simulink model "BMS_Controller"  (R2025b)
settings: Solver=FixedStepDiscrete  StartTime=0.0  StopTime=10.0  FixedStep=Ts  RelTol=1e-3
InitFcn:
  | init_BMS
undefined symbols (not defined in the file): I_charge_OC_release_A, I_charge_OC_trip_A, I_discharge_OC_release_A, I_discharge_OC_trip_A, Q_est_cell_Ah, SOC0_est_pack, T_charge_high_release_C, T_charge_high_trip_C, T_charge_low_release_C, T_charge_low_trip_C, T_discharge_high_release_C, T_discharge_high_trip_C, T_discharge_low_release_C, T_discharge_low_trip_C, Ts, V_cell_OV_release_V, V_cell_OV_trip_V, V_cell_UV_release_V, V_cell_UV_trip_V
libraries: simulink x7
settings Model: Creator=Khadija  LastModifiedBy=Khadija
settings OptimizationCC: DefaultParameterBehavior=Inlined  EnhancedBackFolding=on  PassReuseOutputArgsAs=Individual arguments  ZeroExternalMemoryAtStartup=off  ZeroInternalMemoryAtStartup=off  OptimizeBlockOrder=speed  DifferentSizesBufferReuse=on  OptimizationCustomize=off  EfficientTunableParamExpr=on
settings DebuggingCC: ParameterTunabilityLossMsg=error
settings SFSimCC: MATLABDynamicMemAlloc=off
settings RTWCC: SystemTargetFile=ert.tlc  TemplateMakefile=ert_default_tmf  Description=Embedded Coder
settings CodeAppCC: ForceParamTrailComments=on  IgnoreCustomStorageClasses=off  OperatorAnnotations=on  SimulinkDataObjDesc=on  SFDataObjDesc=on  InsertBlockDesc=on
settings ERTTargetCC: ERTCustomFileTemplate=example_file_process.tlc  TargetLangStandard=C99 (ISO)  GenerateSampleERTMain=on

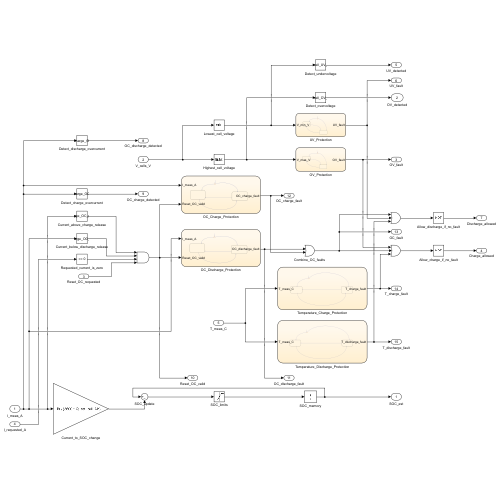
[thumbnail: Simulink's stored preview of the top-level diagram]
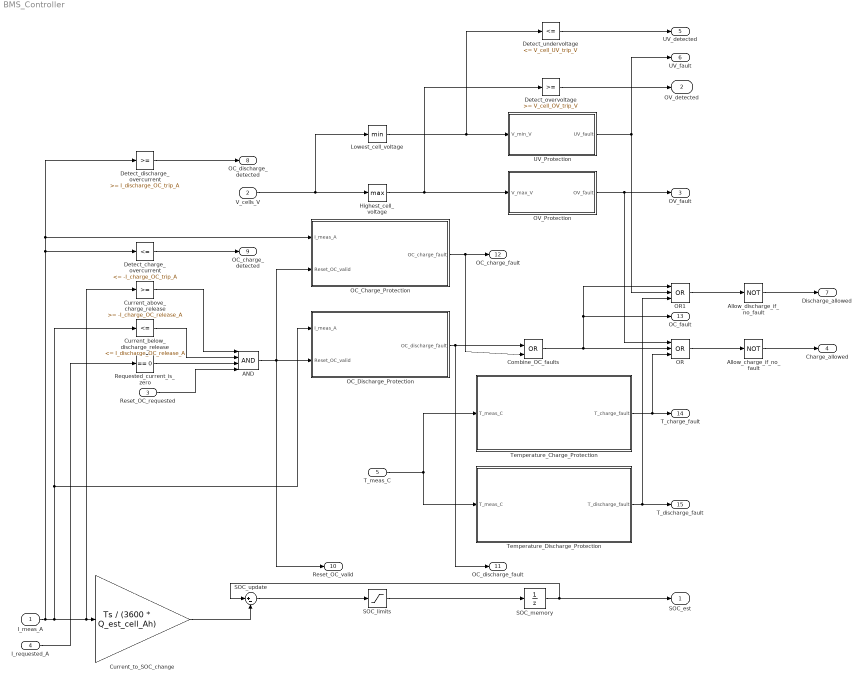
== system BMS_Controller ==
  I_meas_A : Inport
  V_cells_V : Inport  Port=2  OutDataTypeStr=double  PortDimensions=96  SampleTime=Ts
  Reset_OC_requested : Inport  Port=3  OutDataTypeStr=boolean
  I_requested_A : Inport  Port=4  OutDataTypeStr=double
  T_meas_C : Inport  Port=5  OutDataTypeStr=double
  AND : Logic  Inputs=4  IconShape=distinctive  AllPortsSameDT=off  OutDataTypeStr=boolean
  Allow_charge_if_no_fault : Logic  Operator=NOT  AllPortsSameDT=off  OutDataTypeStr=boolean
  Allow_discharge_if_no_fault : Logic  Operator=NOT  AllPortsSameDT=off  OutDataTypeStr=boolean
  Combine_OC_faults : Logic  Operator=OR  IconShape=distinctive  AllPortsSameDT=off  OutDataTypeStr=boolean
  Current_above_charge_release : simulink/Logic and Bit Operations/Compare To Constant  relop=>=  const=-I_charge_OC_release_A  OutDataTypeStr=boolean
  Current_below_discharge_release : simulink/Logic and Bit Operations/Compare To Constant  relop=<=  const=I_discharge_OC_release_A  OutDataTypeStr=boolean
  Current_to_SOC_change : Gain  Gain=Ts / (3600 * Q_est_cell_Ah)
  Detect_charge_overcurrent : simulink/Logic and Bit Operations/Compare To Constant  relop=<=  const=-I_charge_OC_trip_A  OutDataTypeStr=boolean
  Detect_discharge_overcurrent : simulink/Logic and Bit Operations/Compare To Constant  relop=>=  const=I_discharge_OC_trip_A  OutDataTypeStr=boolean
  Detect_overvoltage : simulink/Logic and Bit Operations/Compare To Constant  relop=>=  const=V_cell_OV_trip_V  OutDataTypeStr=boolean
  Detect_undervoltage : simulink/Logic and Bit Operations/Compare To Constant  relop=<=  const=V_cell_UV_trip_V  OutDataTypeStr=boolean
  Highest_cell_voltage : MinMax  Function=max
  Lowest_cell_voltage : MinMax
  OC_Charge_Protection : Stateflow chart  TreatAsAtomicUnit=on
  OC_Discharge_Protection : Stateflow chart  TreatAsAtomicUnit=on
  OR : Logic  Operator=OR  Inputs=3  IconShape=distinctive  AllPortsSameDT=off  OutDataTypeStr=boolean
  OR1 : Logic  Operator=OR  Inputs=3  IconShape=distinctive  AllPortsSameDT=off  OutDataTypeStr=boolean
  OV_Protection : Stateflow chart  TreatAsAtomicUnit=on
  Requested_current_is_zero : simulink/Logic and Bit Operations/Compare To Constant  relop===  const=0  OutDataTypeStr=boolean
  SOC_limits : Saturate  UpperLimit=1  LowerLimit=0
  SOC_memory : UnitDelay  InitialCondition=SOC0_est_pack  SampleTime=Ts  HasFrameUpgradeWarning=on
  SOC_update : Sum  Inputs=|+-
  Temperature_Charge_Protection : Stateflow chart  TreatAsAtomicUnit=on
  Temperature_Discharge_Protection : Stateflow chart  TreatAsAtomicUnit=on
  UV_Protection : Stateflow chart  TreatAsAtomicUnit=on
  SOC_est : Outport
  OV_detected : Outport  Port=2
  OV_fault : Outport  Port=3
  Charge_allowed : Outport  Port=4
  UV_detected : Outport  Port=5
  UV_fault : Outport  Port=6
  Discharge_allowed : Outport  Port=7
  "OC_discharge_detected " : Outport  Port=8  OutDataTypeStr=boolean
  OC_charge_detected : Outport  Port=9  OutDataTypeStr=boolean
  Reset_OC_valid : Outport  Port=10
  OC_discharge_fault : Outport  Port=11
  OC_charge_fault : Outport  Port=12
  OC_fault : Outport  Port=13
  T_charge_fault : Outport  Port=14
  T_discharge_fault : Outport  Port=15
  wires:
  Reset_OC_requested/1 -> AND/4
  I_requested_A/1 -> Requested_current_is_zero/1
  Allow_charge_if_no_fault/1 -> Charge_allowed/1
  I_meas_A/1 -> Current_to_SOC_change/1, Current_above_charge_release/1, Current_below_discharge_release/1, OC_Discharge_Protection/1(I_meas_A), OC_Charge_Protection/1(I_meas_A), Detect_discharge_overcurrent/1, Detect_charge_overcurrent/1
  Current_below_discharge_release/1 -> AND/2
  Lowest_cell_voltage/1 -> UV_Protection/1(V_min_V), Detect_undervoltage/1
  Current_above_charge_release/1 -> AND/1
  Detect_charge_overcurrent/1 -> OC_charge_detected/1
  OC_Charge_Protection/1(OC_charge_fault) -> Combine_OC_faults/2, OC_charge_fault/1
  Detect_discharge_overcurrent/1 -> "OC_discharge_detected "/1
  Requested_current_is_zero/1 -> AND/3
  Current_to_SOC_change/1 -> SOC_update/2
  AND/1 -> Reset_OC_valid/1, OC_Discharge_Protection/2(Reset_OC_valid), OC_Charge_Protection/2(Reset_OC_valid)
  V_cells_V/1 -> Highest_cell_voltage/1, Lowest_cell_voltage/1
  SOC_update/1 -> SOC_limits/1
  Combine_OC_faults/1 -> OR1/1, OC_fault/1, OR/2
  Highest_cell_voltage/1 -> OV_Protection/1(V_max_V), Detect_overvoltage/1
  OC_Discharge_Protection/1(OC_discharge_fault) -> Combine_OC_faults/1, OC_discharge_fault/1
  SOC_limits/1 -> SOC_memory/1
  Detect_undervoltage/1 -> UV_detected/1
  Detect_overvoltage/1 -> OV_detected/1
  UV_Protection/1(UV_fault) -> UV_fault/1, OR1/2
  OV_Protection/1(OV_fault) -> OV_fault/1, OR/1
  Temperature_Charge_Protection/1(T_charge_fault) -> OR/3, T_charge_fault/1
  Temperature_Discharge_Protection/1(T_discharge_fault) -> OR1/3, T_discharge_fault/1
  SOC_memory/1 -> SOC_update/1, SOC_est/1
  OR1/1 -> Allow_discharge_if_no_fault/1
  OR/1 -> Allow_charge_if_no_fault/1
  Allow_discharge_if_no_fault/1 -> Discharge_allowed/1
  T_meas_C/1 -> Temperature_Charge_Protection/1(T_meas_C), Temperature_Discharge_Protection/1(T_meas_C)

== stateflow chart BMS_Controller/Temperature_Charge_Protection ==
  settings: updateMethod=DISCRETE  sampleTime=Ts
  state Normal
    entry:
    T_charge_fault = false;
  state Temperature_fault
    entry:
    T_charge_fault = true;
  (junction 4) -> Temperature_fault [order 1] : [T_meas_C <= T_charge_low_trip_C || T_meas_C >= T_charge_high_trip_C]
  (default) -> (junction 4)
  (junction 4) -> Normal [order 2]
  Temperature_fault -> Normal : [T_meas_C >= T_charge_low_release_C && T_meas_C <= T_charge_high_release_C]
  Normal -> Temperature_fault : [T_meas_C <= T_charge_low_trip_C || T_meas_C >= T_charge_high_trip_C]
  data: T_meas_C input double size=1; T_charge_fault output boolean size=1 =false; T_charge_high_release_C parameter double size=1; T_charge_high_trip_C parameter double size=1; T_charge_low_release_C parameter double size=1; T_charge_low_trip_C parameter double size=1

== stateflow chart BMS_Controller/Temperature_Discharge_Protection ==
  settings: updateMethod=DISCRETE  sampleTime=Ts
  state Normal
    entry:
    T_discharge_fault = false;
  state Temperature_fault
    entry:
    T_discharge_fault = true;
  (junction 4) -> Temperature_fault [order 1] : [T_meas_C <= T_discharge_low_trip_C || T_meas_C >= T_discharge_high_trip_C]
  (default) -> (junction 4)
  (junction 4) -> Normal [order 2]
  Temperature_fault -> Normal : [T_meas_C >= T_discharge_low_release_C && T_meas_C <= T_discharge_high_release_C]
  Normal -> Temperature_fault : [T_meas_C <= T_discharge_low_trip_C || T_meas_C >= T_discharge_high_trip_C]
  data: T_meas_C input double size=1; T_discharge_fault output boolean size=1 =false; T_discharge_high_trip_C parameter double size=1; T_discharge_low_trip_C parameter double size=1; T_discharge_high_release_C parameter double size=1; T_discharge_low_release_C parameter double size=1

== stateflow chart BMS_Controller/UV_Protection ==
  settings: updateMethod=DISCRETE  sampleTime=Ts
  state Normal
    entry:
    UV_fault = false;
  state Overvoltage
    entry:
    UV_fault = true;
  (default) -> (junction 31)
  (junction 31) -> Normal [order 2]
  (junction 31) -> Overvoltage [order 1] : [V_min_V <= V_cell_UV_trip_V]
  Normal -> Overvoltage : [V_min_V <= V_cell_UV_trip_V]
  Overvoltage -> Normal : [V_min_V >= V_cell_UV_release_V]
  data: UV_fault output boolean size=1 =false; V_min_V input double size=1; V_cell_UV_trip_V parameter double size=1; V_cell_UV_release_V parameter double size=1

== stateflow chart BMS_Controller/OC_Discharge_Protection ==
  state Normal
    entry:
    OC_discharge_fault = false;
  state Overcurrent
    entry:
    OC_discharge_fault = true;
  (default) -> (junction 8)
  (junction 8) -> Overcurrent [order 1] : [I_meas_A >= I_discharge_OC_trip_A]
  (junction 8) -> Normal [order 2]
  Overcurrent -> Normal : [Reset_OC_valid]
  Normal -> Overcurrent : [I_meas_A >= I_discharge_OC_trip_A]
  data: I_meas_A input double size=1; Reset_OC_valid input boolean size=1; OC_discharge_fault output boolean size=1; I_discharge_OC_trip_A parameter double size=1

== stateflow chart BMS_Controller/OV_Protection ==
  settings: updateMethod=DISCRETE  sampleTime=Ts
  state Normal
    entry:
    OV_fault = false;
  state Overvoltage
    entry:
    OV_fault = true;
  (default) -> (junction 31)
  (junction 31) -> Normal [order 2]
  (junction 31) -> Overvoltage [order 1] : [V_max_V >= V_cell_OV_trip_V]
  Normal -> Overvoltage : [V_max_V >= V_cell_OV_trip_V]
  Overvoltage -> Normal : [V_max_V <= V_cell_OV_release_V]
  data: OV_fault output boolean size=1 =false; V_max_V input double size=1; V_cell_OV_trip_V parameter double size=1; V_cell_OV_release_V parameter double size=1

== stateflow chart BMS_Controller/OC_Charge_Protection ==
  state Normal
    entry:
    OC_charge_fault = false;
  state Overcurrent
    entry:
    OC_charge_fault = true;
  (default) -> (junction 8)
  (junction 8) -> Overcurrent [order 1] : [I_meas_A <= -I_charge_OC_trip_A]
  (junction 8) -> Normal [order 2]
  Overcurrent -> Normal : [Reset_OC_valid]
  Normal -> Overcurrent : [I_meas_A <= -I_charge_OC_trip_A]
  data: I_meas_A input double size=1; Reset_OC_valid input boolean size=1; OC_charge_fault output boolean size=1; I_charge_OC_trip_A parameter double size=1
